simulink model "boost_frest_diffeq"  (R2025a)
settings: Solver=ode23tb  StartTime=0.0  StopTime=0.5  MaxStep=5e-06  RelTol=1e-05
PreLoadFcn:
  | if ~exist('BM', 'var'), boost_mrac_params; end
InitFcn:
  | if ~exist('BM', 'var'), boost_mrac_params; end
undefined symbols (not defined in the file): BM
libraries: simulink x1
Description:
  | Duty-to-output plant for frestimate (Section II-A of Yanarates & Zhou 2022).
settings Model: Creator=runner  LastModifiedBy=runner
settings DataIOCC: SaveOutput=off  SignalLogging=off  SaveTime=off
settings DebuggingCC: AlgebraicLoopMsg=error

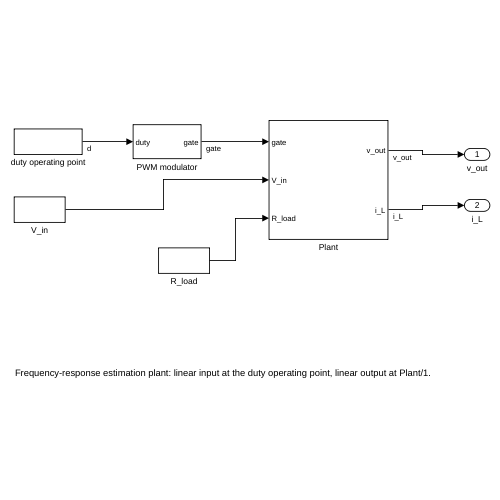
[thumbnail: Simulink's stored preview of the top-level diagram]
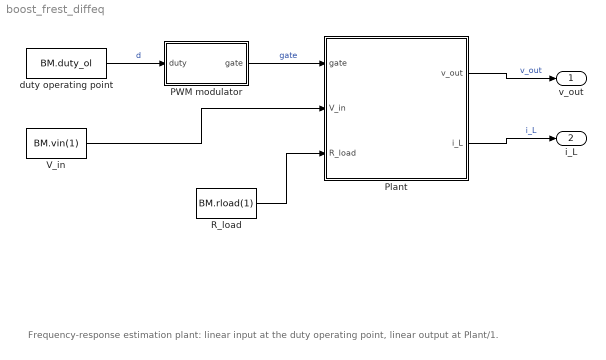
== system boost_frest_diffeq ==
  note: Frequency-response estimation plant: linear input at the duty operating point, linear output at Plant/1.
  PWM modulator : Subsystem
  Plant : Subsystem
  R_load : Constant  Value=BM.rload(1)
  V_in : Constant  Value=BM.vin(1)
  duty operating point : Constant  Value=BM.duty_ol
  v_out : Outport
  i_L : Outport  Port=2
  wires:
  duty operating point/1 -> PWM modulator/1(duty)  "d"
  R_load/1 -> Plant/3(R_load)
  PWM modulator/1(gate) -> Plant/1(gate)  "gate"
  V_in/1 -> Plant/2(V_in)
  Plant/1(v_out) -> v_out/1  "v_out"
  Plant/2(i_L) -> i_L/1  "i_L"

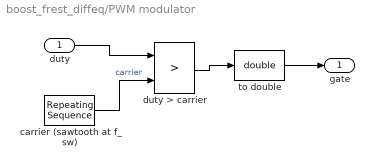
== system boost_frest_diffeq/PWM modulator ==
  duty : Inport
  carrier (sawtooth at f_sw) : simulink/Sources/Repeating Sequence  rep_seq_t=[0 BM.Tsw]  rep_seq_y=[0 1]
  duty > carrier : RelationalOperator  Operator=>  OutDataTypeStr=boolean  RndMeth=Simplest  InputSameDT=off
  to double : DataTypeConversion  OutDataTypeStr=double  SaturateOnIntegerOverflow=off  RndMeth=Floor
  gate : Outport
  wires:
  duty/1 -> duty > carrier/1
  carrier (sawtooth at f_sw)/1 -> duty > carrier/2  "carrier"
  duty > carrier/1 -> to double/1
  to double/1 -> gate/1

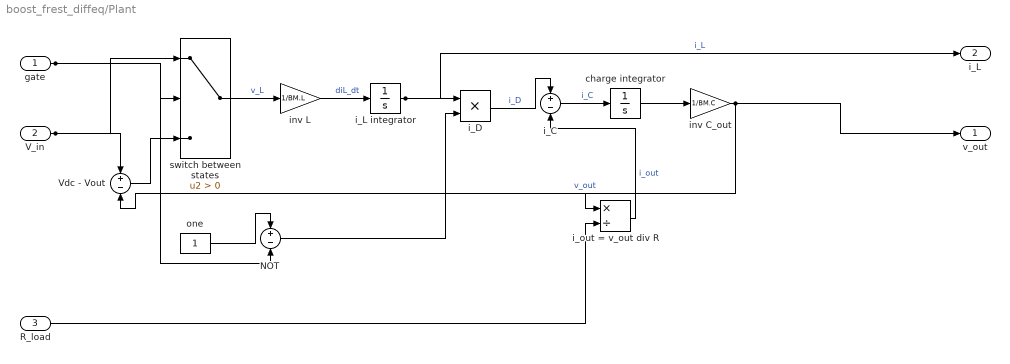
== system boost_frest_diffeq/Plant ==
  gate : Inport
  V_in : Inport  Port=2
  R_load : Inport  Port=3
  NOT : Sum  Inputs=+-
  Vdc - Vout : Sum  Inputs=+-
  charge integrator : Integrator  InitialCondition=BM.C*BM.v0
  i_C : Sum  Inputs=+-
  i_D : Product  Inputs=**
  i_L integrator : Integrator  InitialCondition=BM.iL0  LimitOutput=on  LowerSaturationLimit=BM.iL_min
  i_out = v_out div R : Product  Inputs=*/
  inv C_out : Gain  Gain=1/BM.C
  inv L : Gain  Gain=1/BM.L
  one : Constant
  switch between states : Switch  Criteria=u2 > Threshold  SaturateOnIntegerOverflow=off  InputSameDT=off
  v_out : Outport
  i_L : Outport  Port=2
  wires:
  V_in/1 -> switch between states/1, Vdc - Vout/1
  gate/1 -> switch between states/2, NOT/2
  Vdc - Vout/1 -> switch between states/3
  switch between states/1 -> inv L/1  "v_L"
  inv L/1 -> i_L integrator/1  "diL_dt"
  i_L integrator/1 -> i_D/1, i_L/1  "i_L"
  one/1 -> NOT/1
  NOT/1 -> i_D/2
  i_D/1 -> i_C/1  "i_D"
  i_out = v_out div R/1 -> i_C/2  "i_out"
  i_C/1 -> charge integrator/1  "i_C"
  charge integrator/1 -> inv C_out/1
  inv C_out/1 -> v_out/1, Vdc - Vout/2, i_out = v_out div R/1  "v_out"
  R_load/1 -> i_out = v_out div R/2
